simulink model "DDMR_Simscape_SS_Motor_HBridge"  (R2024b)
settings: Solver=ode23t  StartTime=0.0  StopTime=30  FixedStep=0.005  RelTol=1e-3
values from neighbouring files (symbols this model uses):
  A_steer = [0, -V_ref; 0, 0]    [LQR.m]    (also in Track.m; Track2.m)
  B_steer = [0; 1]    [LQR.m]    (also in Track.m; Track2.m)
  K = lqr(A_full, B_full, Q_lqr, R_lqr)    [LQR.m]    (also in Track.m = [K_brake, 0, 0; Track2.m)
  L = 0.2    [LQR.m]    (also in Track.m; Track2.m)
  L_f = 0.2    [LQR.m]    (also in Track.m; Track2.m)
  L_obs = lqr(A_steer', C_steer', Q_obs, R_obs)'    [LQR.m]    (also in Track.m = place(A_steer', C_steer', poles_obs)'; Track2.m)
  line_width = 0.03    [LQR.m]    (also in Track.m; Track2.m)
  N = size(pts, 1)    [Track2.m]
  R = 0.05    [LQR.m]    (also in Track.m; Track2.m)
  track_pts = [2*cos(linspace(0, 2*pi, 1000)'), 2*sin(linspace(0, 2*pi, 1000)').*cos(linspace(0, 2*pi, 1000)')]    [LQR.m]    (also in Track.m; Track2.m = [track_pts; segments{i}])
  W_spread = 0.15    [LQR.m]    (also in Track.m; Track2.m)
undefined symbols (not defined in the file or in its folder): X, Y, Z
libraries: sm_lib x22, fl_lib x15, nesl_utility x10, ee_lib x6, simulink x2, slpidlib x2, batteryecm_lib x1
(part 2 of 2)

== matlab function DDMR_Simscape_SS_Motor_HBridge/6-Sensor Array1 ==
  data: x input; sensor_readings output; y input; theta input; track_pts input; L_f input; W_spread input; threshold input; sensor_pos output
function [sensor_readings, sensor_pos] = fcn(x, y, theta, track_pts, L_f, W_spread, threshold)
    % 6 sensors spread linearly across the front
    y_offsets = linspace(W_spread/2, -W_spread/2, 6);
    S_loc = [L_f * ones(1,6); y_offsets];
    
    R = [cos(theta), -sin(theta); sin(theta), cos(theta)];
    
    sensor_pos = zeros(2, 6);
    sensor_readings = zeros(1, 6);
    
    for i = 1:6
        % Calculate global position of each sensor
        sensor_pos(:, i) = [x; y] + R * S_loc(:, i);
        
        % Check distance to the track
        dists = sqrt((track_pts(:,1) - sensor_pos(1, i)).^2 + (track_pts(:,2) - sensor_pos(2, i)).^2);
        if min(dists) <= threshold
            sensor_readings(i) = 1;
        end
    end
end

== matlab function DDMR_Simscape_SS_Motor_HBridge/Inverse_Kinematiks 1 ==
  data: v input; omega_L output; omega input; R input; L input; omega_R output
function [omega_L, omega_R] = inverse_kinematics(v, omega, R, L)
    % Calculate linear velocity of each wheel (m/s)
    v_L = v - (omega * L / 2);
    v_R = v + (omega * L / 2);

    % Convert linear velocity to angular velocity (rad/s)
    omega_L = v_L / R;
    omega_R = v_R / R;
end

== matlab function DDMR_Simscape_SS_Motor_HBridge/MATLAB Function2 ==
  settings: updateMethod=DISCRETE
  data: sensor_readings input; e_y output
function e_y = calculate_error(sensor_readings)
    % Physical distances of each sensor from the center of the chassis (in meters)
    % Array total width = 0.15m (+/- 0.075m)
    weights = [0.075, 0.045, 0.015, -0.015, -0.045, -0.075]; 
    
    % Calculate physical lateral error (e_y) in meters
    if sum(sensor_readings) == 0
        e_y = 0; % Maintain heading if no line is detected
    else
        e_y = sum(sensor_readings .* weights);
    end
end
